simulink model "control_invers"  (R2025b)
settings: Solver=VariableStepAuto  StartTime=0.0  StopTime=10.0  RelTol=1e-3
settings Model: Creator=bogdu  LastModifiedBy=Sficaro

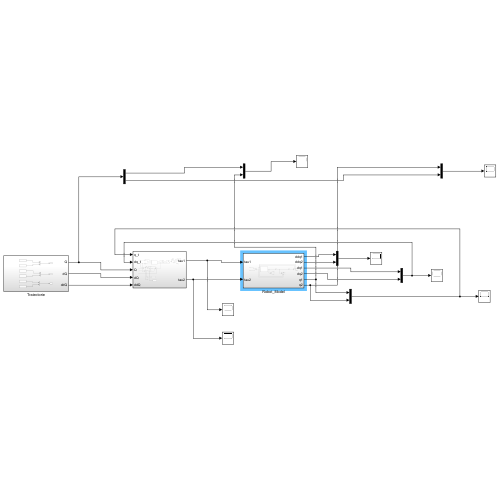
[thumbnail: Simulink's stored preview of the top-level diagram]
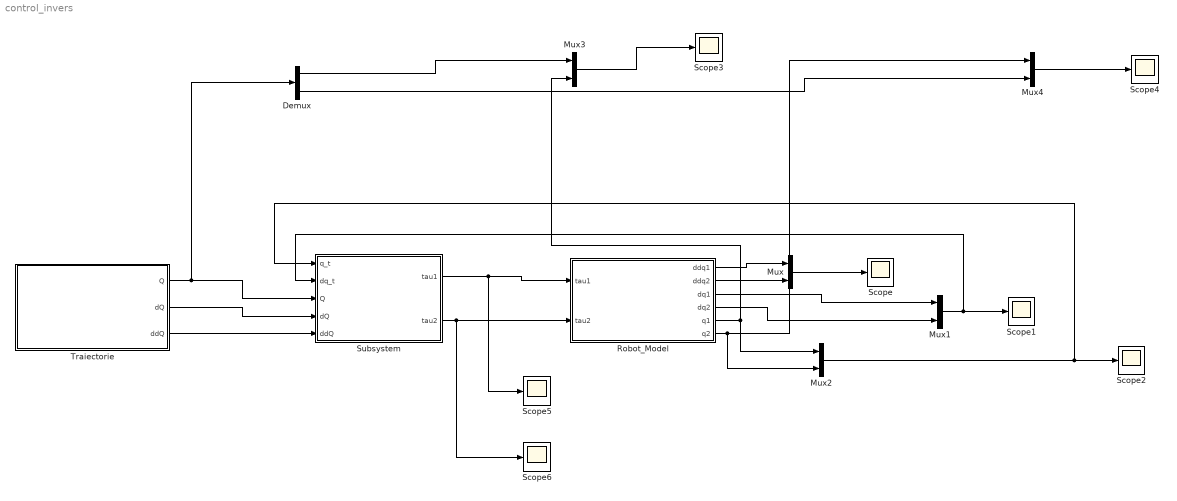
== system control_invers ==
  Demux : Demux  Outputs=2
  Mux{,1..4} (5 alike) : Mux  Inputs=2
  Robot_Model : Subsystem
  Scope{,1..6} (7 alike) : Scope
      Scope settings: ActiveDisplayYMinimum=-0.11705  ActiveDisplayYMaximum=0.11773  DataLoggingVariableName=ScopeData3
      Scope1 settings: ActiveDisplayYMinimum=-0.02951  ActiveDisplayYMaximum=0.26506  DataLoggingVariableName=ScopeData4
      Scope2 settings: ActiveDisplayYMinimum=-0.19629  ActiveDisplayYMaximum=1.76661  DataLoggingVariableName=ScopeData5
      Scope3 settings: ActiveDisplayYMinimum=-0.19635  ActiveDisplayYMaximum=1.76715  DataLoggingVariableName=ScopeData6
      Scope4 settings: ActiveDisplayYMinimum=-0.0125  ActiveDisplayYMaximum=0.1125  DataLoggingVariableName=ScopeData7
      Scope5 settings: ActiveDisplayYMinimum=-0.45146  ActiveDisplayYMaximum=3.89246  DataLoggingVariableName=ScopeData8
      Scope6 settings: ActiveDisplayYMinimum=-0.60938  ActiveDisplayYMaximum=5.51443  DataLoggingVariableName=ScopeData9
  Subsystem : Subsystem
  Traiectorie : Subsystem
  wires:
  Subsystem/1(tau1) -> Scope5/1, Robot_Model/1(tau1)
  Subsystem/2(tau2) -> Scope6/1, Robot_Model/2(tau2)
  Robot_Model/1(ddq1) -> Mux/1
  Robot_Model/2(ddq2) -> Mux/2
  Mux/1 -> Scope/1
  Robot_Model/3(dq1) -> Mux1/1
  Robot_Model/4(dq2) -> Mux1/2
  Traiectorie/3(ddQ) -> Subsystem/5(ddQ)
  Traiectorie/2(dQ) -> Subsystem/4(dQ)
  Traiectorie/1(Q) -> Demux/1, Subsystem/3(Q)
  Mux1/1 -> Scope1/1, Subsystem/2(dq_t)
  Robot_Model/5(q1) -> Mux3/2, Mux2/1
  Robot_Model/6(q2) -> Mux2/2, Mux4/1
  Mux2/1 -> Scope2/1, Subsystem/1(q_t)
  Demux/1 -> Mux3/1
  Mux3/1 -> Scope3/1
  Demux/2 -> Mux4/2
  Mux4/1 -> Scope4/1

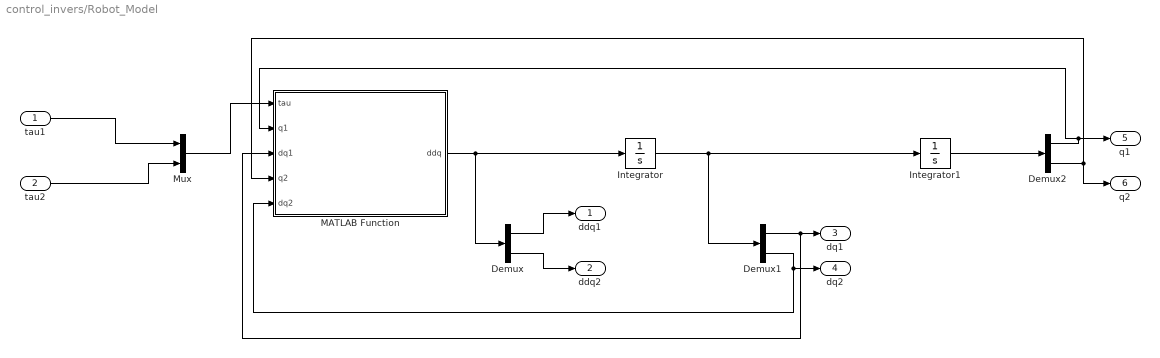
== system control_invers/Robot_Model ==
  tau1 : Inport
  tau2 : Inport  Port=2
  Demux : Demux  Outputs=2
  Demux1 : Demux  Outputs=2
  Demux2 : Demux  Outputs=2
  Integrator : Integrator
  Integrator1 : Integrator
  MATLAB Function : MATLAB Function  TreatAsAtomicUnit=on
  Mux : Mux  Inputs=2
  ddq1 : Outport
  ddq2 : Outport  Port=2
  dq1 : Outport  Port=3
  dq2 : Outport  Port=4
  q1 : Outport  Port=5
  q2 : Outport  Port=6
  wires:
  tau1/1 -> Mux/1
  tau2/1 -> Mux/2
  Mux/1 -> MATLAB Function/1(tau)
  MATLAB Function/1(ddq) -> Integrator/1, Demux/1
  Demux/1 -> ddq1/1
  Demux/2 -> ddq2/1
  Integrator/1 -> Integrator1/1, Demux1/1
  Demux1/1 -> MATLAB Function/3(dq1), dq1/1
  Demux1/2 -> MATLAB Function/5(dq2), dq2/1
  Integrator1/1 -> Demux2/1
  Demux2/1 -> MATLAB Function/2(q1), q1/1
  Demux2/2 -> q2/1, MATLAB Function/4(q2)

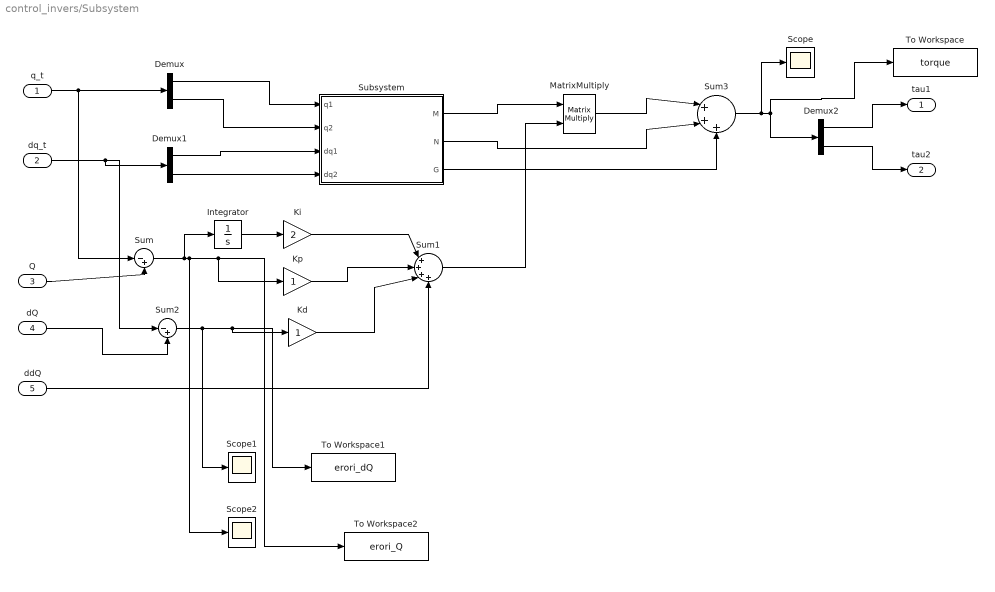
== system control_invers/Subsystem ==
  q_t : Inport
  dq_t : Inport  Port=2
  Q : Inport  Port=3
  dQ : Inport  Port=4
  ddQ : Inport  Port=5
  Demux : Demux  Outputs=2
  Demux1 : Demux  Outputs=2
  Demux2 : Demux  Outputs=2
  Integrator : Integrator
  Kd : Gain
  Ki : Gain  Gain=2
  Kp : Gain
  MatrixMultiply : Product  Multiplication=Matrix(*)
  Scope : Scope
      settings: ActiveDisplayYMinimum=-0.63195950525982769  ActiveDisplayYMaximum=5.51693621163801
  Scope1 : Scope
      settings: ActiveDisplayYMinimum=-0.00029231927860072851  ActiveDisplayYMaximum=0.00045502443619145974
  Scope2 : Scope
      settings: ActiveDisplayYMinimum=-0.00029175549333509965  ActiveDisplayYMaximum=0.000566566772920496  DataLoggingVariableName=ScopeData2
  Subsystem : Subsystem
  Sum : Sum  Inputs=|-+
  Sum1 : Sum  Inputs=|++++
  Sum2 : Sum  Inputs=|-+
  Sum3 : Sum  Inputs=|+++
  To Workspace : ToWorkspace  VariableName=torque  SaveFormat=Timeseries  SampleTime=-1
  To Workspace1 : ToWorkspace  VariableName=erori_dQ  SaveFormat=Timeseries  SampleTime=-1
  To Workspace2 : ToWorkspace  VariableName=erori_Q  SaveFormat=Timeseries  SampleTime=-1
  tau1 : Outport
  tau2 : Outport  Port=2
  wires:
  q_t/1 -> Sum/1, Demux/1
  Demux/1 -> Subsystem/1(q1)
  Demux/2 -> Subsystem/2(q2)
  dq_t/1 -> Sum2/1, Demux1/1
  Demux1/1 -> Subsystem/3(dq1)
  Demux1/2 -> Subsystem/4(dq2)
  Q/1 -> Sum/2
  Integrator/1 -> Ki/1
  Sum/1 -> To Workspace2/1, Kp/1, Scope2/1, Integrator/1
  Ki/1 -> Sum1/1
  Kp/1 -> Sum1/2
  dQ/1 -> Sum2/2
  Sum2/1 -> To Workspace1/1, Kd/1, Scope1/1
  Kd/1 -> Sum1/3
  ddQ/1 -> Sum1/4
  Subsystem/1(M) -> MatrixMultiply/1
  Sum1/1 -> MatrixMultiply/2
  MatrixMultiply/1 -> Sum3/1
  Subsystem/2(N) -> Sum3/2
  Subsystem/3(G) -> Sum3/3
  Sum3/1 -> To Workspace/1, Demux2/1, Scope/1
  Demux2/1 -> tau1/1
  Demux2/2 -> tau2/1

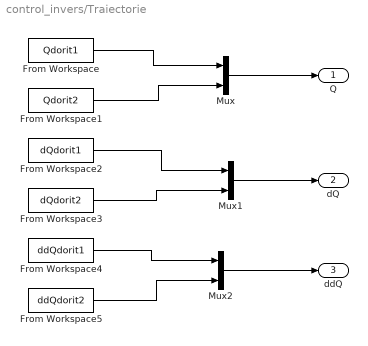
== system control_invers/Traiectorie ==
  From Workspace : FromWorkspace  VariableName=Qdorit1
  From Workspace1 : FromWorkspace  VariableName=Qdorit2
  From Workspace2 : FromWorkspace  VariableName=dQdorit1
  From Workspace3 : FromWorkspace  VariableName=dQdorit2
  From Workspace4 : FromWorkspace  VariableName=ddQdorit1
  From Workspace5 : FromWorkspace  VariableName=ddQdorit2
  Mux : Mux  Inputs=2
  Mux1 : Mux  Inputs=2
  Mux2 : Mux  Inputs=2
  Q : Outport
  dQ : Outport  Port=2
  ddQ : Outport  Port=3
  wires:
  From Workspace/1 -> Mux/1
  From Workspace1/1 -> Mux/2
  From Workspace2/1 -> Mux1/1
  From Workspace3/1 -> Mux1/2
  From Workspace4/1 -> Mux2/1
  From Workspace5/1 -> Mux2/2
  Mux/1 -> Q/1
  Mux1/1 -> dQ/1
  Mux2/1 -> ddQ/1

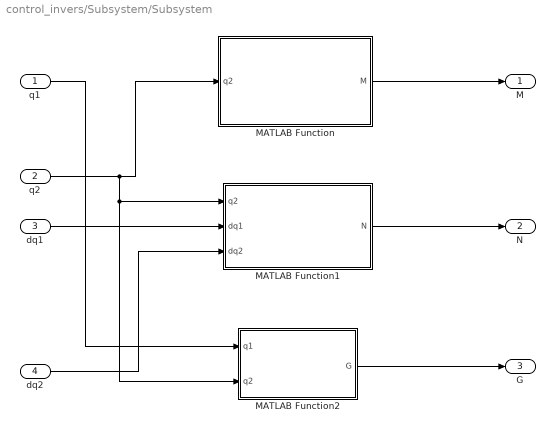
== system control_invers/Subsystem/Subsystem ==
  q1 : Inport
  q2 : Inport  Port=2
  dq1 : Inport  Port=3
  dq2 : Inport  Port=4
  MATLAB Function : MATLAB Function  TreatAsAtomicUnit=on
  MATLAB Function1 : MATLAB Function  TreatAsAtomicUnit=on
  MATLAB Function2 : MATLAB Function  TreatAsAtomicUnit=on
  M : Outport
  N : Outport  Port=2
  G : Outport  Port=3
  wires:
  q2/1 -> MATLAB Function1/1(q2), MATLAB Function2/2(q2), MATLAB Function/1(q2)
  MATLAB Function/1(M) -> M/1
  dq1/1 -> MATLAB Function1/2(dq1)
  dq2/1 -> MATLAB Function1/3(dq2)
  MATLAB Function1/1(N) -> N/1
  q1/1 -> MATLAB Function2/1(q1)
  MATLAB Function2/1(G) -> G/1

== matlab function control_invers/Subsystem/Subsystem/MATLAB Function1 ==
  data: q2 input; N output; dq1 input; dq2 input
function N = n_fct(q2, dq1, dq2)

    mc1 = 0.5;      
    mc2 = 0.5;      
    l1 = 0.4;
    lc2 = 0.1;
    lc1 = 0.2;
    Izz1 = 0.000625;
    Izz2 = 0.00197;
    Ixx_1 = Izz1;
    Ixx_2 = Izz2;
    g=9.81;

    % coriolis
    B_coriolis = [2*mc2*(l1 + lc2 + q2); 
                           0];
    
    % centrifugal
    Cn = [           0,                      0; 
         -mc2*(l1 + lc2 + q2),                0];
    % coriolis + centrifugal
    N = Cn*[dq1^2; dq2^2] + B_coriolis*dq1*dq2;

== matlab function control_invers/Subsystem/Subsystem/MATLAB Function ==
  data: q2 input; M output
function M = M_inertia(q2)

    mc1 = 0.5;      
    mc2 = 0.5;      
    l1 = 0.4;
    lc2 = 0.1;
    lc1 = 0.2;
    Izz1 = 0.000625;
    Izz2 = 0.00197;
    Ixx_1 = Izz1;
    Ixx_2 = Izz2;

    M = [mc2*l1^2 + 2*mc2*l1*lc2 + 2*mc2*l1*q2 + mc1*lc1^2 + mc2*lc2^2 + 2*mc2*lc2*q2 + mc2*q2^2 + Ixx_1 + Ixx_2,              0;
                                                  0,                                                                           mc2];

end

== matlab function control_invers/Subsystem/Subsystem/MATLAB Function2 ==
  data: q1 input; G output; q2 input
function G = gravitatie(q1, q2)

    mc1 = 0.5;      
    mc2 = 0.5;      
    l1 = 0.4;
    lc2 = 0.1;
    lc1 = 0.2;
    Izz1 = 0.000625;
    Izz2 = 0.00197;
    Ixx_1 = Izz1;
    Ixx_2 = Izz2;
    g=9.81;

     G = [g*mc2*(cos(q1)*(l1 + q2) + lc2*cos(q1)) + g*lc1*mc1*cos(q1); 
                               g*mc2*sin(q1)];

== matlab function control_invers/Robot_Model/MATLAB Function ==
  data: tau input; q1 input; ddq output; dq1 input; q2 input; dq2 input
function ddq = calcul_ddq(tau, q1,dq1, q2, dq2)
    
    % parametri structura
    mc1 = 0.5;      
    mc2 = 0.5;      
    l1 = 0.4;
    lc2 = 0.1;
    lc1 = 0.2;
    Izz1 = 0.000625;
    Izz2 = 0.00197;
    % deoarece in Simulink miscarea se face mereu pe z, vom egala momentele
    % de inertie cu cele de pe axa z
    Ixx_1 = Izz1;
    Ixx_2 = Izz2;
    g=9.81;
   
    % mass inertia
    M = [mc2*l1^2 + 2*mc2*l1*lc2 + 2*mc2*l1*q2 + mc1*lc1^2 + mc2*lc2^2 + 2*mc2*lc2*q2 + mc2*q2^2 + Ixx_1 + Ixx_2,              0;
                                                  0,                                                                           mc2];
    

     % coriolis
    B_coriolis = [2*mc2*(l1 + lc2 + q2); 
                           0];
    
    % centrifugal
    Cn = [           0,                      0; 
         -mc2*(l1 + lc2 + q2),                0];
    % coriolis + centrifugal
    N = Cn*[dq1^2; dq2^2] + B_coriolis*dq1*dq2;

    G = [g*mc2*(cos(q1)*(l1 + q2) + lc2*cos(q1)) + g*lc1*mc1*cos(q1); 
                               g*mc2*sin(q1)];

    ddq = inv(M) * (tau - N - G);
